simulink model "AE200_LGS_Model"  (R2021b)
settings: Solver=VariableStepAuto  StartTime=0.0  StopTime=10.0  RelTol=1e-3
InitFcn:
  | LGS_Init
settings Model: Creator=amazgrace  LastModifiedBy=amazgrace

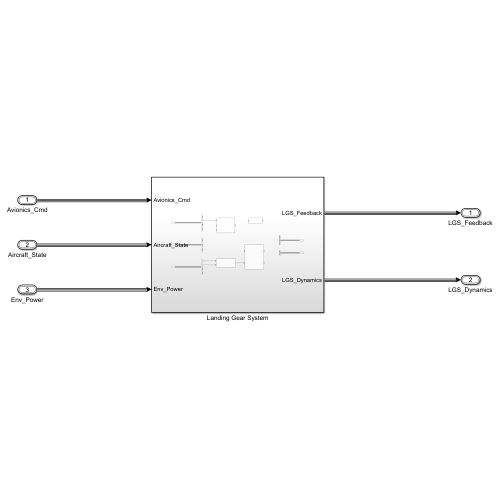
[thumbnail: Simulink's stored preview of the top-level diagram]
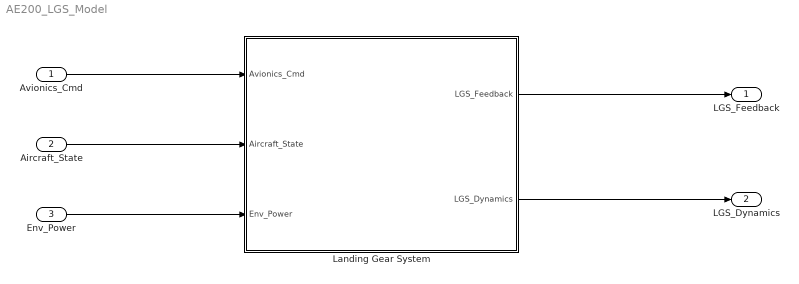
== system AE200_LGS_Model ==
  Avionics_Cmd : Inport  OutDataTypeStr=Bus: Bus_Avionics_In
  Aircraft_State : Inport  Port=2  OutDataTypeStr=Bus: Bus_Aircraft_State
  Env_Power : Inport  Port=3  OutDataTypeStr=Bus: Bus_Env_Power
  Landing Gear System : Subsystem
  LGS_Feedback : Outport  OutDataTypeStr=Bus: Bus_LGS_Feedback
  LGS_Dynamics : Outport  Port=2  OutDataTypeStr=Bus: Bus_LGS_Dynamics
  wires:
  Avionics_Cmd/1 -> Landing Gear System/1(Avionics_Cmd)
  Aircraft_State/1 -> Landing Gear System/2(Aircraft_State)
  Env_Power/1 -> Landing Gear System/3(Env_Power)
  Landing Gear System/1(LGS_Feedback) -> LGS_Feedback/1
  Landing Gear System/2(LGS_Dynamics) -> LGS_Dynamics/1

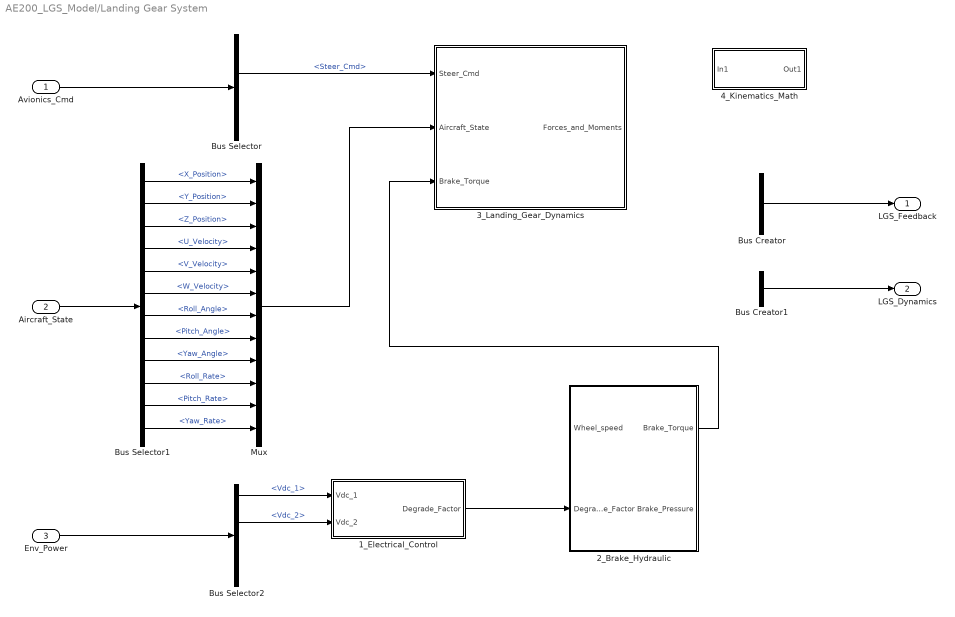
== system AE200_LGS_Model/Landing Gear System ==
  Avionics_Cmd : Inport
  Aircraft_State : Inport  Port=2
  Env_Power : Inport  Port=3
  1_Electrical_Control : Subsystem
  2_Brake_Hydraulic : Subsystem
  3_Landing_Gear_Dynamics : Subsystem
  4_Kinematics_Math : Subsystem
  Bus Creator : BusCreator  Inputs=5
  Bus Creator1 : BusCreator  Inputs=2
  Bus Selector : BusSelector  OutputSignals=Brake_Cmd,Steer_Cmd,Channel_Select,BIT_Trigger
  Bus Selector1 : BusSelector  OutputSignals=X_Position,Y_Position,Z_Position,U_Velocity,V_Velocity,W_Velocity,Roll_Angle,Pitch_Angle,Yaw_Angle,Roll_Rate,Pitch_Rate,Yaw_Rate
  Bus Selector2 : BusSelector  OutputSignals=Vdc_1,Vdc_2,Mu_Ground,Theta_Runway
  Mux : Mux  Inputs=12
  LGS_Feedback : Outport
  LGS_Dynamics : Outport  Port=2
  wires:
  Aircraft_State/1 -> Bus Selector1/1
  Env_Power/1 -> Bus Selector2/1
  Avionics_Cmd/1 -> Bus Selector/1
  Bus Creator1/1 -> LGS_Dynamics/1
  Bus Creator/1 -> LGS_Feedback/1
  Bus Selector2/1 -> 1_Electrical_Control/1(Vdc_1)  "<Vdc_1>"
  Bus Selector2/2 -> 1_Electrical_Control/2(Vdc_2)  "<Vdc_2>"
  1_Electrical_Control/1(Degrade_Factor) -> 2_Brake_Hydraulic/2(Degrade_Factor)
  Bus Selector/2 -> 3_Landing_Gear_Dynamics/1(Steer_Cmd)  "<Steer_Cmd>"
  Bus Selector1/1 -> Mux/1  "<X_Position>"
  Bus Selector1/2 -> Mux/2  "<Y_Position>"
  Bus Selector1/3 -> Mux/3  "<Z_Position>"
  Bus Selector1/4 -> Mux/4  "<U_Velocity>"
  Bus Selector1/5 -> Mux/5  "<V_Velocity>"
  Bus Selector1/6 -> Mux/6  "<W_Velocity>"
  Bus Selector1/7 -> Mux/7  "<Roll_Angle>"
  Bus Selector1/8 -> Mux/8  "<Pitch_Angle>"
  Bus Selector1/9 -> Mux/9  "<Yaw_Angle>"
  Bus Selector1/10 -> Mux/10  "<Roll_Rate>"
  Bus Selector1/11 -> Mux/11  "<Pitch_Rate>"
  Bus Selector1/12 -> Mux/12  "<Yaw_Rate>"
  Mux/1 -> 3_Landing_Gear_Dynamics/2(Aircraft_State)
  2_Brake_Hydraulic/1(Brake_Torque) -> 3_Landing_Gear_Dynamics/3(Brake_Torque)

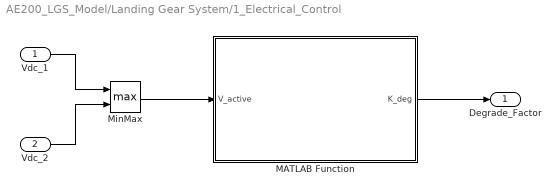
== system AE200_LGS_Model/Landing Gear System/1_Electrical_Control ==
  Vdc_1 : Inport
  Vdc_2 : Inport  Port=2
  MATLAB Function : MATLAB Function  TreatAsAtomicUnit=on
  MinMax : MinMax  Function=max  Inputs=2
  Degrade_Factor : Outport
  wires:
  Vdc_1/1 -> MinMax/1
  Vdc_2/1 -> MinMax/2
  MinMax/1 -> MATLAB Function/1(V_active)
  MATLAB Function/1(K_deg) -> Degrade_Factor/1

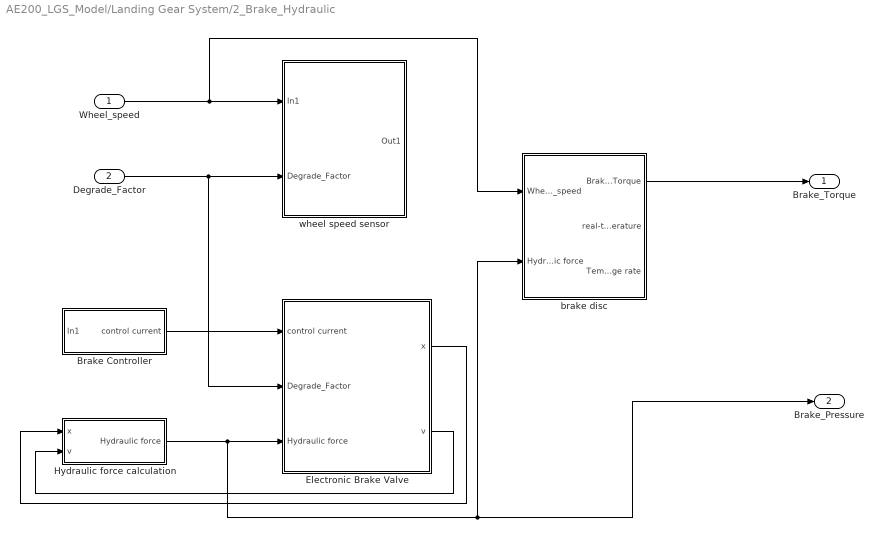
== system AE200_LGS_Model/Landing Gear System/2_Brake_Hydraulic ==
  Wheel_speed : Inport
  Degrade_Factor : Inport  Port=2
  Brake Controller : Subsystem
  Electronic Brake Valve : Subsystem
  Hydraulic force calculation : Subsystem
  brake disc : Subsystem
  wheel speed sensor : Subsystem
  Brake_Torque : Outport
  Brake_Pressure : Outport  Port=2
  wires:
  Degrade_Factor/1 -> Electronic Brake Valve/2(Degrade_Factor), wheel speed sensor/2(Degrade_Factor)
  Wheel_speed/1 -> brake disc/1(Wheel_speed), wheel speed sensor/1(In1)
  Brake Controller/1(control current) -> Electronic Brake Valve/1(control current)
  Hydraulic force calculation/1(Hydraulic force) -> Brake_Pressure/1, brake disc/2(Hydraulic force), Electronic Brake Valve/3(Hydraulic force)
  Electronic Brake Valve/1(x) -> Hydraulic force calculation/1(x)
  Electronic Brake Valve/2(v) -> Hydraulic force calculation/2(v)
  brake disc/1(Brake_Torque) -> Brake_Torque/1

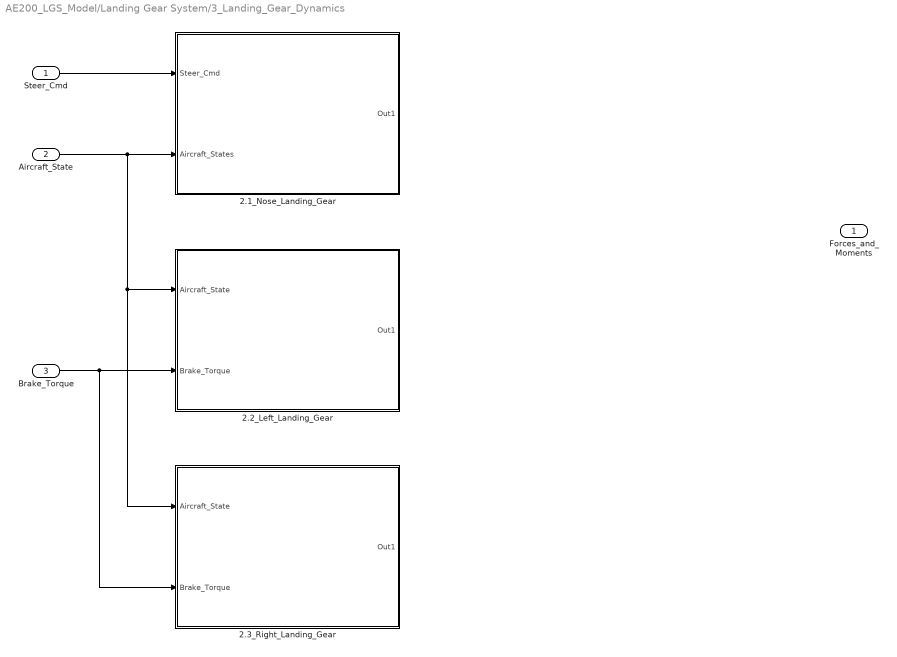
== system AE200_LGS_Model/Landing Gear System/3_Landing_Gear_Dynamics ==
  Steer_Cmd : Inport
  Aircraft_State : Inport  Port=2
  Brake_Torque : Inport  Port=3
  2.1_Nose_Landing_Gear : Subsystem
  2.2_Left_Landing_Gear : Subsystem
  2.3_Right_Landing_Gear : Subsystem
  Forces_and_Moments : Outport
  wires:
  Steer_Cmd/1 -> 2.1_Nose_Landing_Gear/1(Steer_Cmd)
  Aircraft_State/1 -> 2.3_Right_Landing_Gear/1(Aircraft_State), 2.2_Left_Landing_Gear/1(Aircraft_State), 2.1_Nose_Landing_Gear/2(Aircraft_States)
  Brake_Torque/1 -> 2.3_Right_Landing_Gear/2(Brake_Torque), 2.2_Left_Landing_Gear/2(Brake_Torque)

== system AE200_LGS_Model/Landing Gear System/4_Kinematics_Math ==
  In1 : Inport
  Out1 : Outport
  wires:
  In1/1 -> Out1/1

== system AE200_LGS_Model/Landing Gear System/2_Brake_Hydraulic/Brake Controller ==
  In1 : Inport
  control current : Outport
  wires:
  In1/1 -> control current/1

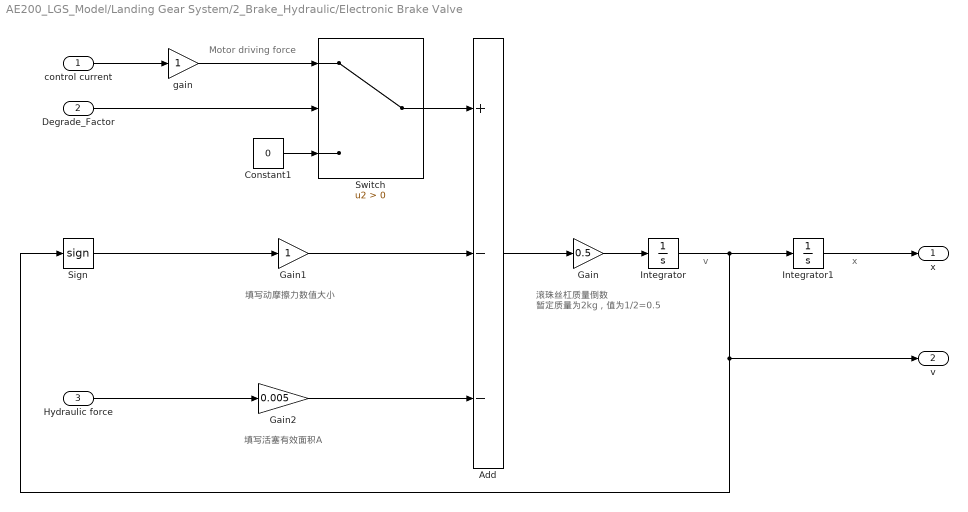
== system AE200_LGS_Model/Landing Gear System/2_Brake_Hydraulic/Electronic Brake Valve ==
  note: Motor driving force
  note: 滚珠丝杠质量倒数
      | 暂定质量为2kg，值为1/2=0.5
  note: v
  note: 填写动摩擦力数值大小
  note: 填写活塞有效面积A
  note: x
  control current : Inport
  Degrade_Factor : Inport  Port=2
  Hydraulic force : Inport  Port=3
  Add : Sum  Inputs=+--
  Constant1 : Constant  Value=0
  Gain : Gain  Gain=0.5
  Gain1 : Gain
  Gain2 : Gain  Gain=0.005
  Integrator : Integrator
  Integrator1 : Integrator
  Sign : Signum
  Switch : Switch  Criteria=u2 > Threshold
  gain : Gain
  x : Outport
  v : Outport  Port=2
  wires:
  control current/1 -> gain/1
  Switch/1 -> Add/1
  gain/1 -> Switch/1
  Constant1/1 -> Switch/3
  Degrade_Factor/1 -> Switch/2
  Add/1 -> Gain/1
  Gain/1 -> Integrator/1
  Integrator/1 -> Integrator1/1, v/1, Sign/1
  Sign/1 -> Gain1/1
  Gain1/1 -> Add/2
  Gain2/1 -> Add/3
  Hydraulic force/1 -> Gain2/1
  Integrator1/1 -> x/1

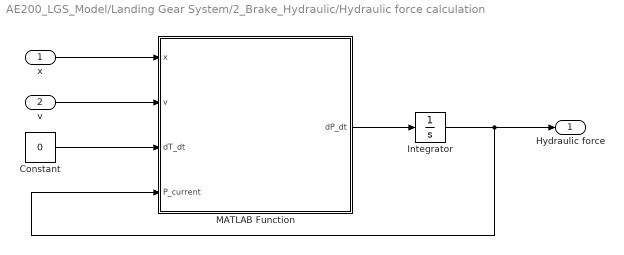
== system AE200_LGS_Model/Landing Gear System/2_Brake_Hydraulic/Hydraulic force calculation ==
  x : Inport
  v : Inport  Port=2
  Constant : Constant  Value=0
  Integrator : Integrator
  MATLAB Function : MATLAB Function  TreatAsAtomicUnit=on
  Hydraulic force : Outport
  wires:
  x/1 -> MATLAB Function/1(x)
  v/1 -> MATLAB Function/2(v)
  MATLAB Function/1(dP_dt) -> Integrator/1
  Integrator/1 -> MATLAB Function/4(P_current), Hydraulic force/1
  Constant/1 -> MATLAB Function/3(dT_dt)

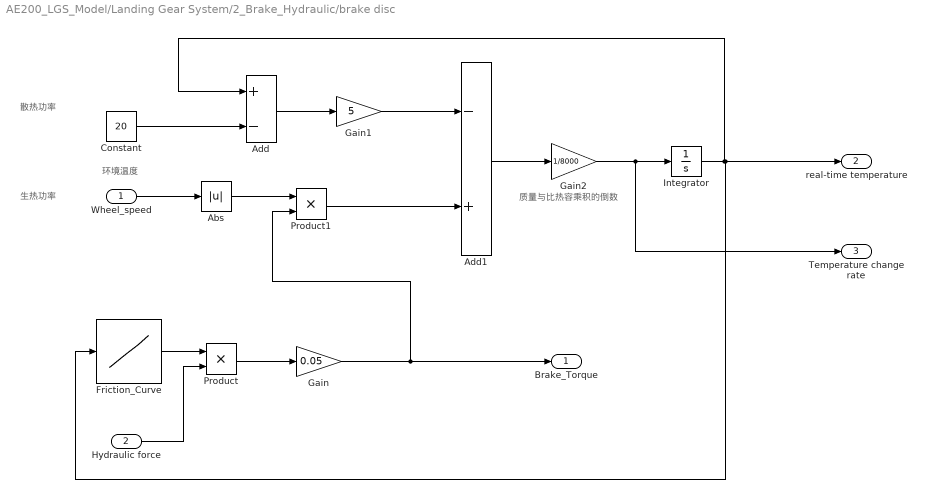
== system AE200_LGS_Model/Landing Gear System/2_Brake_Hydraulic/brake disc ==
  note: 生热功率
  note: 散热功率
  note: 环境温度
  note: 质量与比热容乘积的倒数
  Wheel_speed : Inport
  Hydraulic force : Inport  Port=2
  Abs : Abs
  Add : Sum  Inputs=+-
  Add1 : Sum  Inputs=-+
  Constant : Constant  Value=20
  Friction_Curve : Lookup_n-D  NumberOfTableDimensions=1  BreakpointsForDimension1=[20 100 200 400 600]  Table=[0.35 0.4 0.42 0.38 0.3]  InternalRulePriority=Speed  RndMeth=Simplest  InputSameDT=on
  Gain : Gain  Gain=0.05
  Gain1 : Gain  Gain=5
  Gain2 : Gain  Gain=1/8000
  Integrator : Integrator  InitialCondition=20  LimitOutput=on  UpperSaturationLimit=1000  LowerSaturationLimit=20
  Product : Product
  Product1 : Product
  Brake_Torque : Outport
  real-time temperature : Outport  Port=2
  Temperature change rate : Outport  Port=3
  wires:
  Friction_Curve/1 -> Product/1
  Hydraulic force/1 -> Product/2
  Product/1 -> Gain/1
  Gain/1 -> Product1/2, Brake_Torque/1
  Wheel_speed/1 -> Abs/1
  Abs/1 -> Product1/1
  Constant/1 -> Add/2
  Add/1 -> Gain1/1
  Gain1/1 -> Add1/1
  Product1/1 -> Add1/2
  Add1/1 -> Gain2/1
  Gain2/1 -> Temperature change rate/1, Integrator/1
  Integrator/1 -> real-time temperature/1, Friction_Curve/1, Add/1

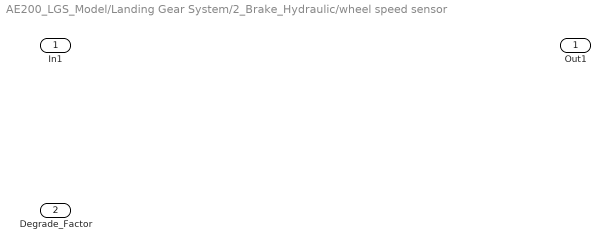
== system AE200_LGS_Model/Landing Gear System/2_Brake_Hydraulic/wheel speed sensor ==
  In1 : Inport
  Degrade_Factor : Inport  Port=2
  Out1 : Outport

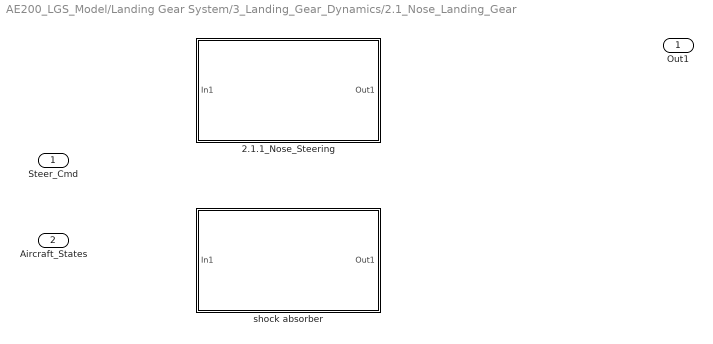
== system AE200_LGS_Model/Landing Gear System/3_Landing_Gear_Dynamics/2.1_Nose_Landing_Gear ==
  Steer_Cmd : Inport
  Aircraft_States : Inport  Port=2
  2.1.1_Nose_Steering : Subsystem
  shock absorber : Subsystem
  Out1 : Outport

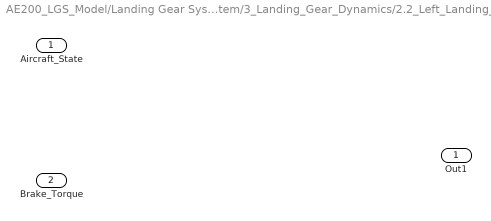
== system AE200_LGS_Model/Landing Gear System/3_Landing_Gear_Dynamics/2.2_Left_Landing_Gear ==
  Aircraft_State : Inport
  Brake_Torque : Inport  Port=2
  Out1 : Outport

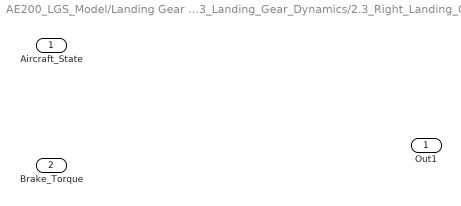
== system AE200_LGS_Model/Landing Gear System/3_Landing_Gear_Dynamics/2.3_Right_Landing_Gear ==
  Aircraft_State : Inport
  Brake_Torque : Inport  Port=2
  Out1 : Outport

== system AE200_LGS_Model/Landing Gear System/3_Landing_Gear_Dynamics/2.1_Nose_Landing_Gear/2.1.1_Nose_Steering ==
  In1 : Inport
  Out1 : Outport
  wires:
  In1/1 -> Out1/1

== system AE200_LGS_Model/Landing Gear System/3_Landing_Gear_Dynamics/2.1_Nose_Landing_Gear/shock absorber ==
  In1 : Inport
  Out1 : Outport
  wires:
  In1/1 -> Out1/1

== matlab function AE200_LGS_Model/Landing Gear System/2_Brake_Hydraulic/Hydraulic force calculation/MATLAB Function ==
  data: x input; dP_dt output; v input; dT_dt input; P_current input
function dP_dt = calculate_pressure_rate(x, v, dT_dt, P_current)
    % 1. 定义常量（根据实际物理参数进行修改）
    B = 1.5e9;        % 体积弹性模量 (Pa)
    V = 0.001;        % 初始容积 (m^3)
    alpha = 7e-4;     % 热膨胀系数 (1/K)
    A_piston = 0.005; % 活塞面积 (m^2)

    % 2. 计算容积变化率 Q2 (与丝杠速度 v 负相关)
    Q2 = -A_piston * v;

    % 3. 计算流入/漏油速率 Q1 
    % （这里需要根据位置 x 或压力判断刹车/回退的补油与漏油状态）
    % 以下为基础逻辑框架，根据具体阀门或泄漏特性微调：
    C_leak = 1e-11; % 假设的泄漏系数
    
    if x < 0.001 
        % 假设 x 小于某个阈值表示退回到了补油孔位置，开启补油机制
        % 具体的补油流量 Q_makeup 需要根据你的系统压力差设定，这里假设为0或常数
        Q1 = 0; 
    else
        % 正常建压刹车状态下，仅考虑因高压产生的微小泄漏（泄漏量与当前压力成正比）
        Q1 = -C_leak * P_current; 
    end

    % 4. 核心公式：计算压力变化率 dP_dt
    % dp/dt = (B/V) * (Q1 + Q2) + alpha * B * (dT/dt)
    dP_dt = (B / V) * (Q1 + Q2) + alpha * B * dT_dt;
end

== matlab function AE200_LGS_Model/Landing Gear System/1_Electrical_Control/MATLAB Function ==
  data: V_active input; K_deg output
function K_deg = fcn(V_active)
    if V_active >= 22.0
        K_deg = 1.0;
    elseif V_active >= 18.0
        K_deg = (V_active - 18.0) / (22.0 - 18.0);
    else
        K_deg = 0.0;
    end
end
